simulink model "original_long_instrumented"  (R2026b)
settings: Solver=ode4  StopTime=4  FixedStep=1.0000000000000001e-05
InitFcn:
  | acf_select_actuator(bdroot);
model workspace (MAT data in the model file):
  acfControlVersion = 'force-observer-v1'
  acfImplementation = 'simple'
  acfLayoutVersion = 1
  p : object (value not decoded)
  pCompliant : object (value not decoded)
  pNearContact : object (value not decoded)
  pNoSprings : object (value not decoded)
  pRecommended : object (value not decoded)
symbols that are objects in the model workspace (value not decoded): p
undefined symbols (not defined in the file): DiscIntNeverNeededParam
(part 2 of 3)

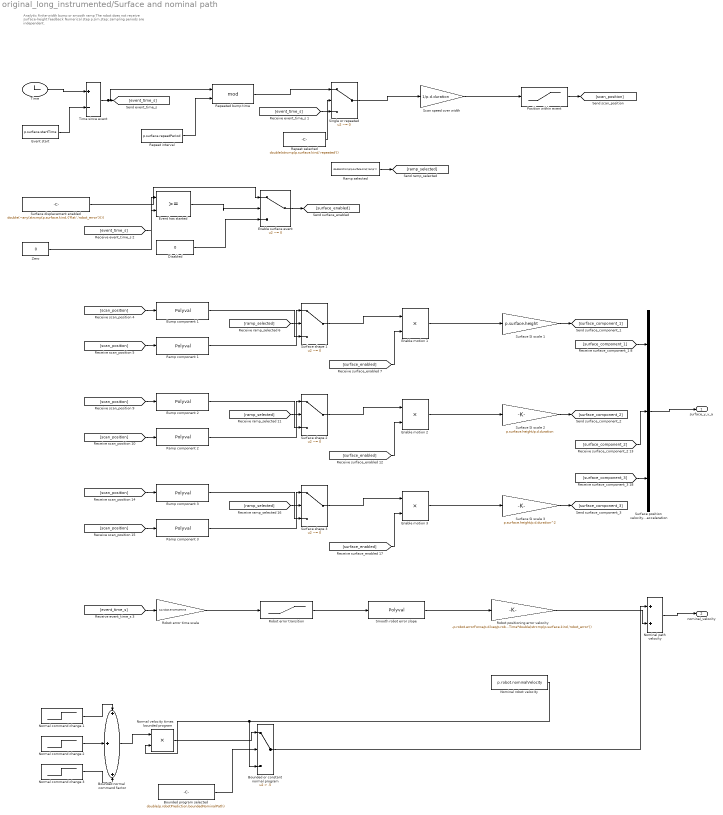
== system original_long_instrumented/Surface and nominal path ==
  note: Analytic finite-width bump or smooth ramp
      | The robot does not receive surface-height feedback
      | Numerical step p.sim.step; sampling periods are independent.
  Bounded normal command factor : Sum  Inputs=+++
  Bounded or constant normal program : Switch  Criteria=u2 > Threshold  Threshold=.5  SaturateOnIntegerOverflow=off  InputSameDT=off
  Bounded program selected : Constant  Value=double(p.robotPrediction.boundedNominalPath)
  Bump component 1 : Polyval  Coefs=[-64 192 -192 64 0 0 0]
  Bump component 2 : Polyval  Coefs=[-384 960 -768 192 0 0]
  Bump component 3 : Polyval  Coefs=[-1920 3840 -2304 384 0]
  Disabled : Constant  Value=0
  Enable motion 1 : Product
  Enable motion 2 : Product
  Enable motion 3 : Product
  Enable surface event : Switch  Criteria=u2 ~= 0  SaturateOnIntegerOverflow=off  InputSameDT=off
  Event has started : RelationalOperator  OutDataTypeStr=boolean  RndMeth=Simplest  InputSameDT=off
  Event start : Constant  Value=p.surface.startTime
  Nominal path velocity : Sum
  Nominal robot velocity : Constant  Value=p.robot.nominalVelocity
  Normal command change 1 : Step  SampleTime=p.robot.sampleTime
  Normal command change 2 : Step  Time=2  FinalValue=-2  SampleTime=p.robot.sampleTime
  Normal command change 3 : Step  Time=3  SampleTime=p.robot.sampleTime
  Normal velocity times bounded program : Product
  Position within event : Saturate  UpperLimit=1  LowerLimit=0
  Ramp component 1 : Polyval  Coefs=[6 -15 10 0 0 0]
  Ramp component 2 : Polyval  Coefs=[30 -60 30 0 0]
  Ramp component 3 : Polyval  Coefs=[120 -180 60 0]
  Ramp selected : Constant  Value=double(strcmp(p.surface.kind,'ramp'))
  Repeat interval : Constant  Value=p.surface.repeatPeriod
  Repeat selected : Constant  Value=double(strcmp(p.surface.kind,'repeated'))
  Repeated bump time : Math  Operator=mod
  Robot error time scale : Gain  Gain=1/p.robot.errorRiseTime
  Robot error transition : Saturate  UpperLimit=1  LowerLimit=0
  Robot positioning error velocity : Gain  Gain=-p.robot.errorForce/p.d.keq/p.robot.errorRiseTime*double(strcmp(p.surface.kind,'robot_error'))
  Scan speed over width : Gain  Gain=1/p.d.duration
  Single or repeated : Switch  Criteria=u2 ~= 0  SaturateOnIntegerOverflow=off  InputSameDT=off
  Smooth robot error slope : Polyval  Coefs=[30 -60 30 0 0]
  Surface SI scale 1 : Gain  Gain=p.surface.height
  Surface SI scale 2 : Gain  Gain=p.surface.height/p.d.duration
  Surface SI scale 3 : Gain  Gain=p.surface.height/p.d.duration^2
  Surface displacement enabled : Constant  Value=double(~any(strcmp(p.surface.kind,{'flat','robot_error'})))
  Surface position velocity acceleration : Mux  Inputs=3
  Surface shape 1 : Switch  Criteria=u2 ~= 0  SaturateOnIntegerOverflow=off  InputSameDT=off
  Surface shape 2 : Switch  Criteria=u2 ~= 0  SaturateOnIntegerOverflow=off  InputSameDT=off
  Surface shape 3 : Switch  Criteria=u2 ~= 0  SaturateOnIntegerOverflow=off  InputSameDT=off
  Time : Clock
  Time since event : Sum  Inputs=+-
  Zero : Constant  Value=0
  surface_y_v_a : Outport
  nominal_velocity : Outport  Port=2
  wires:
  [scan_position] -> Bump component 1/1
  [scan_position] -> Bump component 2/1
  [scan_position] -> Bump component 3/1
  Surface shape 1/1 -> Enable motion 1/1
  [surface_enabled] -> Enable motion 1/2
  Surface shape 2/1 -> Enable motion 2/1
  [surface_enabled] -> Enable motion 2/2
  Surface shape 3/1 -> Enable motion 3/1
  [surface_enabled] -> Enable motion 3/2
  Surface displacement enabled/1 -> Enable surface event/1
  Event has started/1 -> Enable surface event/2
  Disabled/1 -> Enable surface event/3
  [event_time_s] -> Event has started/1
  Zero/1 -> Event has started/2
  Robot positioning error velocity/1 -> Nominal path velocity/2
  Scan speed over width/1 -> Position within event/1
  [scan_position] -> Ramp component 1/1
  [scan_position] -> Ramp component 2/1
  [scan_position] -> Ramp component 3/1
  Time since event/1 -> Repeated bump time/1, [event_time_s]
  Repeat interval/1 -> Repeated bump time/2
  [event_time_s] -> Robot error time scale/1
  Robot error time scale/1 -> Robot error transition/1
  Smooth robot error slope/1 -> Robot positioning error velocity/1
  Single or repeated/1 -> Scan speed over width/1
  Ramp selected/1 -> [ramp_selected]
  Position within event/1 -> [scan_position]
  Surface SI scale 1/1 -> [surface_component_1]
  Surface SI scale 2/1 -> [surface_component_2]
  Surface SI scale 3/1 -> [surface_component_3]
  Enable surface event/1 -> [surface_enabled]
  Repeated bump time/1 -> Single or repeated/1
  Repeat selected/1 -> Single or repeated/2
  [event_time_s] -> Single or repeated/3
  Robot error transition/1 -> Smooth robot error slope/1
  Enable motion 1/1 -> Surface SI scale 1/1
  Enable motion 2/1 -> Surface SI scale 2/1
  Enable motion 3/1 -> Surface SI scale 3/1
  [surface_component_1] -> Surface position velocity acceleration/1
  [surface_component_2] -> Surface position velocity acceleration/2
  [surface_component_3] -> Surface position velocity acceleration/3
  Ramp component 1/1 -> Surface shape 1/1
  [ramp_selected] -> Surface shape 1/2
  Bump component 1/1 -> Surface shape 1/3
  Ramp component 2/1 -> Surface shape 2/1
  [ramp_selected] -> Surface shape 2/2
  Bump component 2/1 -> Surface shape 2/3
  Ramp component 3/1 -> Surface shape 3/1
  [ramp_selected] -> Surface shape 3/2
  Bump component 3/1 -> Surface shape 3/3
  Time/1 -> Time since event/1
  Event start/1 -> Time since event/2
  Surface position velocity acceleration/1 -> surface_y_v_a/1
  Nominal path velocity/1 -> nominal_velocity/1
  Normal command change 1/1 -> Bounded normal command factor/1
  Normal command change 2/1 -> Bounded normal command factor/2
  Normal command change 3/1 -> Bounded normal command factor/3
  Bounded normal command factor/1 -> Normal velocity times bounded program/1
  Nominal robot velocity/1 -> Normal velocity times bounded program/2, Bounded or constant normal program/3
  Normal velocity times bounded program/1 -> Bounded or constant normal program/1
  Bounded program selected/1 -> Bounded or constant normal program/2
  Bounded or constant normal program/1 -> Nominal path velocity/1

== system original_long_instrumented/Surface contact force ==
  Axial reaction : Inport
  Physical surface velocity : Inport  Port=2
  Axial reaction factor : Sum  Inputs=+-
  Friction times slope : Gain  Gain=p.contact.mu
  Lateral reaction : Product  Inputs=**/
  Lateral sign : Gain  Gain=-1
  Normal reaction : Product  Inputs=**/
  Normalizer : Math  Operator=sqrt
  Slope plus friction : Bias  Bias=p.contact.mu  SaturateOnIntegerOverflow=off
  Squared slope : Math  Operator=square
  Squared slope plus one : Bias  Bias=1  SaturateOnIntegerOverflow=off
  Surface slope : Gain  Gain=1/p.surface.scanSpeed
  Unity : Constant
  Velocity component : Selector  InputPortWidth=3  IndexOptions=Index vector (dialog)  Indices=2  OutputSizes=1
  tag scope: actual_contact_slope=global, lateral_contact_N=global, normal_contact_N=global
  wires:
  Physical surface velocity/1 -> Velocity component/1
  Velocity component/1 -> Surface slope/1
  Surface slope/1 -> Squared slope/1, Friction times slope/1, Slope plus friction/1, [actual_contact_slope]
  Squared slope/1 -> Squared slope plus one/1
  Squared slope plus one/1 -> Normalizer/1
  Unity/1 -> Axial reaction factor/1
  Friction times slope/1 -> Axial reaction factor/2
  Axial reaction/1 -> Normal reaction/1
  Normalizer/1 -> Normal reaction/2, Lateral reaction/3
  Axial reaction factor/1 -> Normal reaction/3
  Normal reaction/1 -> Lateral reaction/1, [normal_contact_N]
  Slope plus friction/1 -> Lateral reaction/2
  Lateral reaction/1 -> Lateral sign/1
  Lateral sign/1 -> [lateral_contact_N]

== system original_long_instrumented/Actuator and RABS mechanics/Actuator ==
  Command : Inport
  Gap position velocity : Inport  Port=2
  Spring load : Inport  Port=3
  Ideal position : Subsystem  VariantControl=Ideal position
  Leadscrew : Subsystem  VariantControl=Leadscrew
  Voice coil : Subsystem  VariantControl=Voice coil
  Transmitted force : Outport
  Drive measurements : Outport  Port=2

== system original_long_instrumented/Actuator and RABS mechanics/B to S spring and damper ==
  S position velocity : Inport
  B position velocity : Inport  Port=2
  Rigid reaction : Inport  Port=3
  Compliant or rigid link : VariantSource  VariantControlMode=label  LabelModeActiveChoice=Compliant  VariantControls={Compliant, Rigid}
  Damping : Gain  Gain=p.mechanics.c1
  Endpoint difference : Sum  Inputs=+-
  Preload : Constant  Value=p.d.q10
  Spring and damper force : Sum  Inputs=+++
  Spring displacement and relative velocity : Demux  Outputs=2
  Stiffness : Gain  Gain=p.mechanics.k1
  Spring force : Outport
  wires:
  Spring displacement and relative velocity/2 -> Damping/1
  S position velocity/1 -> Endpoint difference/1
  B position velocity/1 -> Endpoint difference/2
  Preload/1 -> Spring and damper force/1
  Stiffness/1 -> Spring and damper force/2
  Damping/1 -> Spring and damper force/3
  Endpoint difference/1 -> Spring displacement and relative velocity/1
  Spring displacement and relative velocity/1 -> Stiffness/1
  Spring and damper force/1 -> Compliant or rigid link/1
  Rigid reaction/1 -> Compliant or rigid link/2
  Compliant or rigid link/1 -> Spring force/1

== system original_long_instrumented/Actuator and RABS mechanics/Mass A ==
  Actuator force : Inport
  Upper spring force : Inport  Port=2
  Gravity : Constant  Value=p.d.g
  Inverse mass : Gain  Gain=1/p.mechanics.mA
  Net applied force : Sum  Inputs=+-
  Newton acceleration : Sum  Inputs=+-
  Position : Integrator  InitialCondition=p.d.u0
  Position and velocity : Mux  Inputs=2
  Velocity : Integrator
  Position velocity : Outport
  Acceleration : Outport  Port=2
  wires:
  Net applied force/1 -> Inverse mass/1
  Actuator force/1 -> Net applied force/1
  Upper spring force/1 -> Net applied force/2
  Inverse mass/1 -> Newton acceleration/1
  Gravity/1 -> Newton acceleration/2
  Velocity/1 -> Position/1, [velocity_m_s]
  Position/1 -> Position and velocity/1
  [velocity_m_s] -> Position and velocity/2
  Newton acceleration/1 -> Velocity/1, Acceleration/1
  Position and velocity/1 -> Position velocity/1

== system original_long_instrumented/Actuator and RABS mechanics/Mass B ==
  Lower spring force : Inport
  Actuator force : Inport  Port=2
  Gravity : Constant  Value=p.d.g
  Inverse mass : Gain  Gain=1/p.mechanics.mB
  Net applied force : Sum  Inputs=+-
  Newton acceleration : Sum  Inputs=+-
  Position : Integrator
  Position and velocity : Mux  Inputs=2
  Velocity : Integrator
  Position velocity : Outport
  Acceleration : Outport  Port=2
  wires:
  Net applied force/1 -> Inverse mass/1
  Lower spring force/1 -> Net applied force/1
  Actuator force/1 -> Net applied force/2
  Inverse mass/1 -> Newton acceleration/1
  Gravity/1 -> Newton acceleration/2
  Velocity/1 -> Position/1, [velocity_m_s]
  Position/1 -> Position and velocity/1
  [velocity_m_s] -> Position and velocity/2
  Newton acceleration/1 -> Velocity/1, Acceleration/1
  Position and velocity/1 -> Position velocity/1

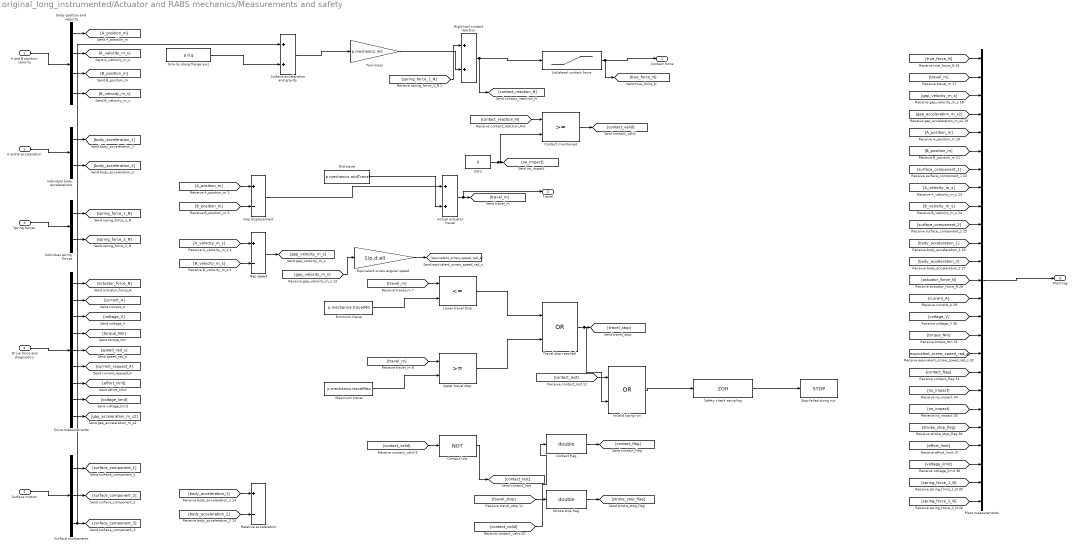
== system original_long_instrumented/Actuator and RABS mechanics/Measurements and safety ==
  A and B position velocity : Inport
  A and B acceleration : Inport  Port=2
  Spring forces : Inport  Port=3
  Drive force and diagnostics : Inport  Port=4
  Surface motion : Inport  Port=5
  Actual actuator travel : Sum
  Body position and velocity : Demux
  Contact flag : DataTypeConversion  OutDataTypeStr=double  SaturateOnIntegerOverflow=off  RndMeth=Floor
  Contact lost : Logic  Operator=NOT  AllPortsSameDT=off  OutDataTypeStr=boolean
  Contact maintained : RelationalOperator  OutDataTypeStr=boolean  RndMeth=Simplest  InputSameDT=off
  Drive measurements : Demux  Outputs=9
  Equivalent screw angular speed : Gain  Gain=1/p.d.ell
  Gap displacement : Sum  Inputs=+-
  Gap speed : Sum  Inputs=+-
  Gravity along flange axis : Constant  Value=p.d.g
  Individual body accelerations : Demux  Outputs=2
  Individual spring forces : Demux  Outputs=2
  Invalid sizing run : Logic  Operator=OR  AllPortsSameDT=off  OutDataTypeStr=boolean
  Lower travel stop : RelationalOperator  Operator=<=  OutDataTypeStr=boolean  RndMeth=Simplest  InputSameDT=off
  Maximum travel : Constant  Value=p.mechanics.travelMax
  Mid travel : Constant  Value=p.mechanics.midTravel
  Minimum travel : Constant  Value=p.mechanics.travelMin
  Plant measurements : Mux  Inputs=25
  Relative acceleration : Sum  Inputs=+-
  Rigid tool contact reaction : Sum
  Safety check sampling : ZeroOrderHold  SampleTime=p.sim.step
  Stop failed sizing run : Stop
  Stroke stop flag : DataTypeConversion  OutDataTypeStr=double  SaturateOnIntegerOverflow=off  RndMeth=Floor
  Surface acceleration and gravity : Sum
  Surface components : Demux  Outputs=3
  Tool mass : Gain  Gain=p.mechanics.mS
  Travel stop reached : Logic  Operator=OR  AllPortsSameDT=off  OutDataTypeStr=boolean
  Unilateral contact force : Saturate  UpperLimit=inf  LowerLimit=0
  Upper travel stop : RelationalOperator  OutDataTypeStr=boolean  RndMeth=Simplest  InputSameDT=off
  Zero : Constant  Value=0
  Contact force : Outport
  Travel : Outport  Port=2
  Plant log : Outport  Port=3
  wires:
  Gap displacement/1 -> Actual actuator travel/1
  Mid travel/1 -> Actual actuator travel/2
  A and B position velocity/1 -> Body position and velocity/1
  [contact_valid] -> Contact flag/1
  [contact_valid] -> Contact lost/1
  [contact_reaction_N] -> Contact maintained/1
  Zero/1 -> Contact maintained/2, [no_impact]
  Drive force and diagnostics/1 -> Drive measurements/1
  [gap_velocity_m_s] -> Equivalent screw angular speed/1
  [A_position_m] -> Gap displacement/1
  [B_position_m] -> Gap displacement/2
  [A_velocity_m_s] -> Gap speed/1
  [B_velocity_m_s] -> Gap speed/2
  A and B acceleration/1 -> Individual body accelerations/1
  Spring forces/1 -> Individual spring forces/1
  [contact_lost] -> Invalid sizing run/1
  Travel stop reached/1 -> Invalid sizing run/2, [travel_stop]
  [travel_m] -> Lower travel stop/1
  Minimum travel/1 -> Lower travel stop/2
  [true_force_N] -> Plant measurements/1
  [travel_m] -> Plant measurements/2
  [gap_velocity_m_s] -> Plant measurements/3
  [gap_acceleration_m_s2] -> Plant measurements/4
  [A_position_m] -> Plant measurements/5
  [B_position_m] -> Plant measurements/6
  [surface_component_1] -> Plant measurements/7
  [A_velocity_m_s] -> Plant measurements/8
  [B_velocity_m_s] -> Plant measurements/9
  [surface_component_2] -> Plant measurements/10
  [body_acceleration_1] -> Plant measurements/11
  [body_acceleration_2] -> Plant measurements/12
  [actuator_force_N] -> Plant measurements/13
  [current_A] -> Plant measurements/14
  [voltage_V] -> Plant measurements/15
  [torque_Nm] -> Plant measurements/16
  [equivalent_screw_speed_rad_s] -> Plant measurements/17
  [contact_flag] -> Plant measurements/18
  [no_impact] -> Plant measurements/19
  [no_impact] -> Plant measurements/20
  [stroke_stop_flag] -> Plant measurements/21
  [effort_limit] -> Plant measurements/22
  [voltage_limit] -> Plant measurements/23
  [spring_force_1_N] -> Plant measurements/24
  [spring_force_2_N] -> Plant measurements/25
  [body_acceleration_1] -> Relative acceleration/1
  [body_acceleration_2] -> Relative acceleration/2
  [spring_force_1_N] -> Rigid tool contact reaction/1
  Tool mass/1 -> Rigid tool contact reaction/2
  Invalid sizing run/1 -> Safety check sampling/1
  Body position and velocity/1 -> [A_position_m]
  Body position and velocity/2 -> [A_velocity_m_s]
  Body position and velocity/3 -> [B_position_m]
  Body position and velocity/4 -> [B_velocity_m_s]
  Drive measurements/1 -> [actuator_force_N]
  Individual body accelerations/1 -> [body_acceleration_1]
  Individual body accelerations/2 -> [body_acceleration_2]
  Contact flag/1 -> [contact_flag]
  Contact lost/1 -> [contact_lost]
  Rigid tool contact reaction/1 -> [contact_reaction_N], Unilateral contact force/1
  Contact maintained/1 -> [contact_valid]
  Drive measurements/2 -> [current_A]
  Drive measurements/6 -> [current_request_A]
  Drive measurements/7 -> [effort_limit]
  Equivalent screw angular speed/1 -> [equivalent_screw_speed_rad_s]
  Drive measurements/9 -> [gap_acceleration_m_s2]
  Gap speed/1 -> [gap_velocity_m_s]
  Drive measurements/5 -> [speed_rad_s]
  Individual spring forces/1 -> [spring_force_1_N]
  Individual spring forces/2 -> [spring_force_2_N]
  Stroke stop flag/1 -> [stroke_stop_flag]
  Surface components/1 -> [surface_component_1]
  Surface components/2 -> [surface_component_2]
  Surface components/3 -> [surface_component_3], Surface acceleration and gravity/1
  Drive measurements/4 -> [torque_Nm]
  Actual actuator travel/1 -> [travel_m], Travel/1
  Unilateral contact force/1 -> [true_force_N], Contact force/1
  Drive measurements/3 -> [voltage_V]
  Drive measurements/8 -> [voltage_limit]
  Safety check sampling/1 -> Stop failed sizing run/1
  [travel_stop] -> Stroke stop flag/1
  Gravity along flange axis/1 -> Surface acceleration and gravity/2
  Surface motion/1 -> Surface components/1
  Surface acceleration and gravity/1 -> Tool mass/1
  Lower travel stop/1 -> Travel stop reached/1
  Upper travel stop/1 -> Travel stop reached/2
  [travel_m] -> Upper travel stop/1
  Maximum travel/1 -> Upper travel stop/2
  Plant measurements/1 -> Plant log/1

== system original_long_instrumented/Actuator and RABS mechanics/R to A spring and damper ==
  A position velocity : Inport
  R position velocity : Inport  Port=2
  Rigid reaction : Inport  Port=3
  Compliant or rigid link : VariantSource  VariantControlMode=label  LabelModeActiveChoice=Rigid  VariantControls={Compliant, Rigid}
  Damping : Gain  Gain=p.mechanics.c2
  Endpoint difference : Sum  Inputs=+-
  Preload : Constant  Value=p.d.q20
  Spring and damper force : Sum  Inputs=+++
  Spring displacement and relative velocity : Demux  Outputs=2
  Stiffness : Gain  Gain=p.mechanics.k2
  Spring force : Outport
  wires:
  Spring displacement and relative velocity/2 -> Damping/1
  A position velocity/1 -> Endpoint difference/1
  R position velocity/1 -> Endpoint difference/2
  Preload/1 -> Spring and damper force/1
  Stiffness/1 -> Spring and damper force/2
  Damping/1 -> Spring and damper force/3
  Endpoint difference/1 -> Spring displacement and relative velocity/1
  Spring displacement and relative velocity/1 -> Stiffness/1
  Spring and damper force/1 -> Compliant or rigid link/1
  Rigid reaction/1 -> Compliant or rigid link/2
  Compliant or rigid link/1 -> Spring force/1

== system original_long_instrumented/Contact force measurement/Contact force reconstruction ==
  raw_cell_error_N : Inport
  Cell error to deviation : Gain  Gain=-1
  Compensated axial reaction : Sum
  Compensated lateral reaction : Sum
  Downstream X inertia : Gain  Gain=p.sensor.distalMass_model_kg
  Downstream Z inertia : Gain  Gain=p.sensor.distalMass_model_kg
  Tared axial cell force : Bias  Bias=p.force.reference  SaturateOnIntegerOverflow=off
  axial_contact_N : Outport
  lateral_contact_N : Outport  Port=2
  tag scope: inertial_axial_contact_N=global, inertial_lateral_contact_N=global
  wires:
  Compensated axial reaction/1 -> axial_contact_N/1, [inertial_axial_contact_N]
  Tared axial cell force/1 -> Compensated axial reaction/1
  Downstream Z inertia/1 -> Compensated axial reaction/2
  Compensated lateral reaction/1 -> lateral_contact_N/1, [inertial_lateral_contact_N]
  Cell error to deviation/1 -> Tared axial cell force/1
  [measured_S_acceleration_z] -> Downstream Z inertia/1
  [measured_lateral_contact_N] -> Compensated lateral reaction/1
  Downstream X inertia/1 -> Compensated lateral reaction/2
  raw_cell_error_N/1 -> Cell error to deviation/1
  [measured_S_acceleration_x] -> Downstream X inertia/1

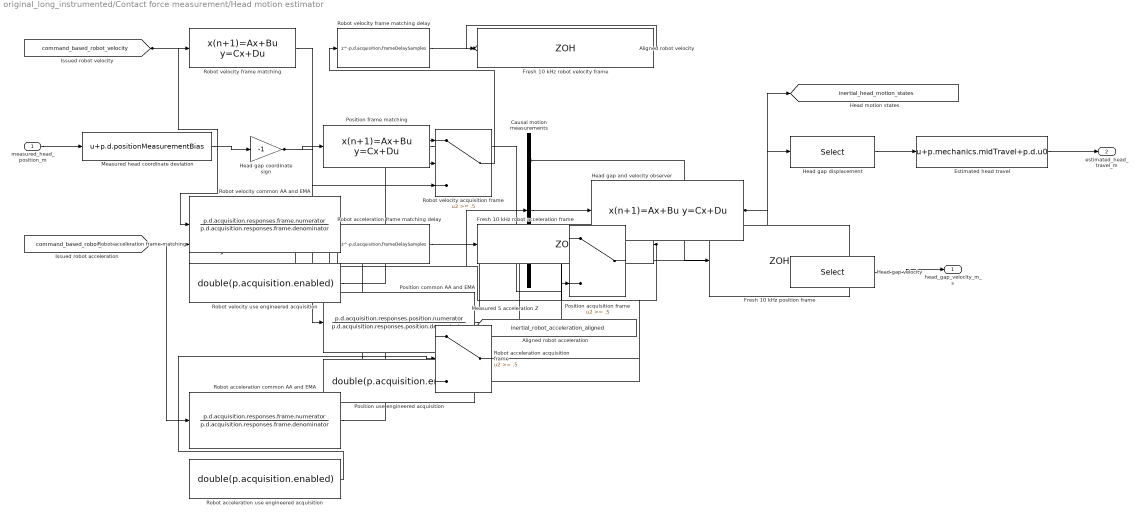
== system original_long_instrumented/Contact force measurement/Head motion estimator ==
  measured_head_position_m : Inport
  Causal motion measurements : Mux  Inputs=3
  Estimated head travel : Bias  Bias=p.mechanics.midTravel+p.d.u0  SaturateOnIntegerOverflow=off
  Fresh 10 kHz position frame : ZeroOrderHold  SampleTime=p.force.sampleTime
  Fresh 10 kHz robot acceleration frame : ZeroOrderHold  SampleTime=p.force.sampleTime
  Fresh 10 kHz robot velocity frame : ZeroOrderHold  SampleTime=p.force.sampleTime
  Head gap and velocity observer : DiscreteStateSpace  A=p.d.toolMotionObserver.A  B=p.d.toolMotionObserver.B  C=p.d.toolMotionObserver.C  D=p.d.toolMotionObserver.D  InitialCondition=zeros(2,1)  SampleTime=p.force.sampleTime
  Head gap coordinate sign : Gain  Gain=-1
  Head gap displacement : Selector  InputPortWidth=2  IndexOptions=Index vector (dialog)  Indices=1  OutputSizes=1
  Head gap velocity : Selector  InputPortWidth=2  IndexOptions=Index vector (dialog)  Indices=2  OutputSizes=1
  Measured head coordinate deviation : Bias  Bias=p.d.positionMeasurementBias  SaturateOnIntegerOverflow=off
  Position acquisition frame : Switch  Threshold=.5  SaturateOnIntegerOverflow=off  InputSameDT=off
  Position common AA and EMA : DiscreteTransferFcn  Numerator=p.d.acquisition.responses.position.numerator  Denominator=p.d.acquisition.responses.position.denominator  InitialStates=(0)*p.d.acquisition.responses.position.steadyStatePerUnitInput  SampleTime=p.sensor.sampleTime
  Position frame matching : DiscreteStateSpace  A=exp(-p.sensor.sampleTime/p.sensor.filterTime)  B=1-exp(-p.sensor.sampleTime/p.sensor.filterTime)  C=exp(-p.sensor.sampleTime/p.sensor.filterTime)  D=1-exp(-p.sensor.sampleTime/p.sensor.filterTime)  SampleTime=p.sensor.sampleTime
  Position use engineered acquisition : Constant  Value=double(p.acquisition.enabled)
  Robot acceleration acquisition frame : Switch  Threshold=.5  SaturateOnIntegerOverflow=off  InputSameDT=off
  Robot acceleration common AA and EMA : DiscreteTransferFcn  Numerator=p.d.acquisition.responses.frame.numerator  Denominator=p.d.acquisition.responses.frame.denominator  InitialStates=(0)*p.d.acquisition.responses.frame.steadyStatePerUnitInput  SampleTime=p.sensor.sampleTime
  Robot acceleration frame matching : DiscreteStateSpace  A=exp(-p.sensor.sampleTime/p.sensor.filterTime)  B=1-exp(-p.sensor.sampleTime/p.sensor.filterTime)  C=exp(-p.sensor.sampleTime/p.sensor.filterTime)  D=1-exp(-p.sensor.sampleTime/p.sensor.filterTime)  SampleTime=p.sensor.sampleTime
  Robot acceleration frame matching delay : Delay  DelayLength=p.d.acquisition.frameDelaySamples  InitialCondition=0  SampleTime=p.sensor.sampleTime
  Robot acceleration use engineered acquisition : Constant  Value=double(p.acquisition.enabled)
  Robot velocity acquisition frame : Switch  Threshold=.5  SaturateOnIntegerOverflow=off  InputSameDT=off
  Robot velocity common AA and EMA : DiscreteTransferFcn  Numerator=p.d.acquisition.responses.frame.numerator  Denominator=p.d.acquisition.responses.frame.denominator  InitialStates=(0)*p.d.acquisition.responses.frame.steadyStatePerUnitInput  SampleTime=p.sensor.sampleTime
  Robot velocity frame matching : DiscreteStateSpace  A=exp(-p.sensor.sampleTime/p.sensor.filterTime)  B=1-exp(-p.sensor.sampleTime/p.sensor.filterTime)  C=exp(-p.sensor.sampleTime/p.sensor.filterTime)  D=1-exp(-p.sensor.sampleTime/p.sensor.filterTime)  SampleTime=p.sensor.sampleTime
  Robot velocity frame matching delay : Delay  DelayLength=p.d.acquisition.frameDelaySamples  InitialCondition=0  SampleTime=p.sensor.sampleTime
  Robot velocity use engineered acquisition : Constant  Value=double(p.acquisition.enabled)
  head_gap_velocity_m_s : Outport
  estimated_head_travel_m : Outport  Port=2
  tag scope: inertial_head_motion_states=global, inertial_robot_acceleration_aligned=global, inertial_robot_velocity_aligned=global
  wires:
  Estimated head travel/1 -> estimated_head_travel_m/1
  measured_head_position_m/1 -> Measured head coordinate deviation/1
  Head gap velocity/1 -> head_gap_velocity_m_s/1
  [command_based_robot_velocity] -> Robot velocity frame matching/1, Robot velocity common AA and EMA/1
  Measured head coordinate deviation/1 -> Head gap coordinate sign/1
  [command_based_robot_acceleration] -> Robot acceleration frame matching/1, Robot acceleration common AA and EMA/1
  Head gap coordinate sign/1 -> Position frame matching/1, Position common AA and EMA/1
  Causal motion measurements/1 -> Head gap and velocity observer/1
  Head gap displacement/1 -> Estimated head travel/1
  Head gap and velocity observer/1 -> Head gap displacement/1, Head gap velocity/1, [inertial_head_motion_states]
  [measured_S_acceleration_z] -> Causal motion measurements/3
  Position common AA and EMA/1 -> Position acquisition frame/1
  Position use engineered acquisition/1 -> Position acquisition frame/2
  Position frame matching/1 -> Position acquisition frame/3
  Position acquisition frame/1 -> Fresh 10 kHz position frame/1
  Fresh 10 kHz position frame/1 -> Causal motion measurements/1
  Robot acceleration common AA and EMA/1 -> Robot acceleration acquisition frame/1
  Robot acceleration use engineered acquisition/1 -> Robot acceleration acquisition frame/2
  Robot acceleration frame matching/1 -> Robot acceleration acquisition frame/3
  Robot acceleration acquisition frame/1 -> Robot acceleration frame matching delay/1
  Robot acceleration frame matching delay/1 -> Fresh 10 kHz robot acceleration frame/1
  Fresh 10 kHz robot acceleration frame/1 -> [inertial_robot_acceleration_aligned], Causal motion measurements/2
  Robot velocity common AA and EMA/1 -> Robot velocity acquisition frame/1
  Robot velocity use engineered acquisition/1 -> Robot velocity acquisition frame/2
  Robot velocity frame matching/1 -> Robot velocity acquisition frame/3
  Robot velocity acquisition frame/1 -> Robot velocity frame matching delay/1
  Robot velocity frame matching delay/1 -> Fresh 10 kHz robot velocity frame/1
  Fresh 10 kHz robot velocity frame/1 -> [inertial_robot_velocity_aligned]

== system original_long_instrumented/Contact force measurement/Normal force projection ==
  Compensated axial force : Inport
  Compensated lateral force : Inport  Port=2
  Head gap velocity : Inport  Port=3
  Axial reference deviation : Bias  Bias=-p.force.reference  SaturateOnIntegerOverflow=off
  Causal surface direction : Gain  Gain=1/p.contact.commandedScanSpeed_m_s
  Estimated S velocity : Sum  Inputs=+-
  Lateral projection : Product  Inputs=**
  Measured drag audit vector : Mux  Inputs=3
  Measured drag geometry : Subsystem
  Measured drag geometry selected : Constant  Value=double(strcmp(p.contact.geometryMode,'measured_drag_ratio'))
  Measured drag native log : ToWorkspace  VariableName=measured_drag_log  SaveFormat=Timeseries  SampleTime=-1
  Measured drag native sample 1 : ZeroOrderHold  SampleTime=p.sim.step
  Measured drag native sample 2 : ZeroOrderHold  SampleTime=p.sim.step
  Measured drag native sample 3 : ZeroOrderHold  SampleTime=p.sim.step
  Measured normal force : Product  Inputs=*/
  Measured normal force deviation : Bias  Bias=-p.force.reference  SaturateOnIntegerOverflow=off
  Normal projection numerator : Sum  Inputs=+-
  Normal reference projection : Gain  Gain=p.force.reference
  Normalizer : Math  Operator=sqrt
  Requested axial force : Sum
  Select axial force geometry request : Switch  Threshold=.5  SaturateOnIntegerOverflow=off  InputSameDT=off
  Squared slope : Math  Operator=square
  Squared slope plus one : Bias  Bias=1  SaturateOnIntegerOverflow=off
  normal_force_deviation_N : Outport
  axial_reference_deviation_N : Outport  Port=2
  tag scope: estimated_contact_slope=global, estimated_normal_contact_N=global, requested_axial_contact_N=global
  wires:
  Axial reference deviation/1 -> axial_reference_deviation_N/1
  Measured normal force deviation/1 -> normal_force_deviation_N/1
  Head gap velocity/1 -> Estimated S velocity/2
  [inertial_robot_velocity_aligned] -> Estimated S velocity/1
  Squared slope/1 -> Squared slope plus one/1
  Compensated lateral force/1 -> Lateral projection/1, Measured drag geometry/2(reconstructed_Rx_N)
  Lateral projection/1 -> Normal projection numerator/2, Requested axial force/2
  Estimated S velocity/1 -> Causal surface direction/1
  Compensated axial force/1 -> Normal projection numerator/1, Measured drag geometry/1(reconstructed_Rz_N)
  Normal reference projection/1 -> Requested axial force/1
  Normal projection numerator/1 -> Measured normal force/1
  Normalizer/1 -> Measured normal force/2, Normal reference projection/1, Measured drag geometry/5(normalizer)
  Causal surface direction/1 -> Squared slope/1, [estimated_contact_slope], Lateral projection/2, Measured drag geometry/3(estimated_slope)
  Squared slope plus one/1 -> Normalizer/1
  Measured normal force/1 -> Measured normal force deviation/1, [estimated_normal_contact_N], Measured drag geometry/4(estimated_normal_N)
  Measured drag geometry/1(requested_Rz_N) -> Select axial force geometry request/1
  Measured drag geometry selected/1 -> Select axial force geometry request/2
  Requested axial force/1 -> Select axial force geometry request/3
  Select axial force geometry request/1 -> Axial reference deviation/1, [requested_axial_contact_N]
  Measured drag geometry/2(filtered_drag_ratio) -> Measured drag native sample 1/1
  Measured drag native sample 1/1 -> Measured drag audit vector/1
  Measured drag geometry/3(bounded_raw_drag_ratio) -> Measured drag native sample 2/1
  Measured drag native sample 2/1 -> Measured drag audit vector/2
  Measured drag geometry/4(drag_estimate_valid) -> Measured drag native sample 3/1
  Measured drag native sample 3/1 -> Measured drag audit vector/3
  Measured drag audit vector/1 -> Measured drag native log/1

== system original_long_instrumented/Force controller/Coil PI and PID ==
  error_N : Inport
  measured_travel_m : Inport  Port=2
  Current limits : Saturate  UpperLimit=p.coil.peakCurrent  LowerLimit=-p.coil.peakCurrent
  Current saturation error : Sum  Inputs=+-
  Flat holding current : Constant  Value=(p.force.reference-(p.uncertainty.massB_model_kg+p.sensor.distalMass_model_kg)*p.d.g)/p.uncertainty.forceConstant_model_N_A
  Integral anti windup : Gain  Gain=-p.force.antiWindupRate/p.inertial.forceKi
  Lower spring inverse feedforward : Subsystem
  Measured motion feedforward : Subsystem
  Normal force PI and PID : Subsystem
  Optional structural-mode current notch : DiscreteTransferFcn  Numerator=p.d.currentNotch.numerator  Denominator=p.d.currentNotch.denominator  InitialStates=p.d.currentNotch.initialStates  SampleTime=p.force.sampleTime
  PI PID and feedforward current : Sum  Inputs=++++++
  command : Outport
  estimated_travel_m : Outport  Port=2
  estimated_force_error_N : Outport  Port=3
  wires:
  measured_travel_m/1 -> estimated_travel_m/1
  Optional structural-mode current notch/1 -> Current limits/1, Current saturation error/2
  Integral anti windup/1 -> Normal force PI and PID/2(anti_windup)
  Current limits/1 -> command/1, Current saturation error/1
  PI PID and feedforward current/1 -> Optional structural-mode current notch/1
  Current saturation error/1 -> Integral anti windup/1
  error_N/1 -> estimated_force_error_N/1, Normal force PI and PID/1(error_N)
  Flat holding current/1 -> PI PID and feedforward current/1
  Normal force PI and PID/1(feedback_current_A) -> PI PID and feedforward current/2
  Measured motion feedforward/1(acceleration_current_A) -> PI PID and feedforward current/3
  Measured motion feedforward/2(geometry_current_A) -> PI PID and feedforward current/4
  Measured motion feedforward/3(friction_current_A) -> PI PID and feedforward current/5
  Lower spring inverse feedforward/1(extra_current_A) -> PI PID and feedforward current/6

== system original_long_instrumented/Force controller/Drive PI and PID ==
  note: Sampled PI + anti-windup
      | Coil: amperes; screw: rad/s; ideal: gap in metres
      | Numerical step p.sim.step; sampling periods are independent.
  note: PI / FILTERED PID
      | Kp, Ki, Kd and derivative-filter time are ordinary parameters.
      | Kd = 0 disables derivative action. Voice-coil strategy chooses this page or the observer.
  error_N : Inport
  measured_travel_m : Inport  Port=2
  Actuator command limits : Saturate  UpperLimit=p.d.commandMax  LowerLimit=p.d.commandMin
  Anti windup : Gain  Gain=p.force.antiWindupRate
  Derivative gain : Gain  Gain=p.d.forceKd*double(strcmp(p.coil.strategy,'pid'))
  Filtered force derivative : DiscreteTransferFcn  Numerator=(1-exp(-p.force.sampleTime/p.d.derivativeFilter))/p.force.sampleTime*[1 -1]  Denominator=[1 -exp(-p.force.sampleTime/p.d.derivativeFilter)]  SampleTime=p.force.sampleTime
  Force controller sampling : ZeroOrderHold  SampleTime=p.force.sampleTime
  Holding command : Constant  Value=p.d.forceFeedforward
  Integral action : DiscreteIntegrator  SampleTime=p.force.sampleTime  ICPrevOutput=DiscIntNeverNeededParam  ICPrevScaledInput=DiscIntNeverNeededParam
  Integral gain : Gain  Gain=p.d.forceKi
  Integral input : Sum
  PI plus holding command : Sum  Inputs=++++
  Proportional gain : Gain  Gain=p.d.forceKp
  Saturation error : Sum  Inputs=+-
  command : Outport
  estimated_travel_m : Outport  Port=2
  estimated_force_error_N : Outport  Port=3
  wires:
  Actuator command limits/1 -> [limited_command], command/1
  Integral action/1 -> [integral_command]
  PI plus holding command/1 -> Actuator command limits/1, [raw_command]
  Integral input/1 -> Integral action/1
  Holding command/1 -> PI plus holding command/3
  error_N/1 -> estimated_force_error_N/1, Force controller sampling/1
  measured_travel_m/1 -> estimated_travel_m/1
  [force_error_N] -> Integral gain/1
  [force_error_N] -> Filtered force derivative/1
  Derivative gain/1 -> [derivative_command]
  Saturation error/1 -> Anti windup/1
  [limited_command] -> Saturation error/1
  Force controller sampling/1 -> Proportional gain/1, [force_error_N]
  Anti windup/1 -> [tracking_correction]
  [raw_command] -> Saturation error/2
  Integral gain/1 -> Integral input/1
  [derivative_command] -> PI plus holding command/4
  [integral_command] -> PI plus holding command/2
  Filtered force derivative/1 -> Derivative gain/1
  [tracking_correction] -> Integral input/2
  Proportional gain/1 -> PI plus holding command/1

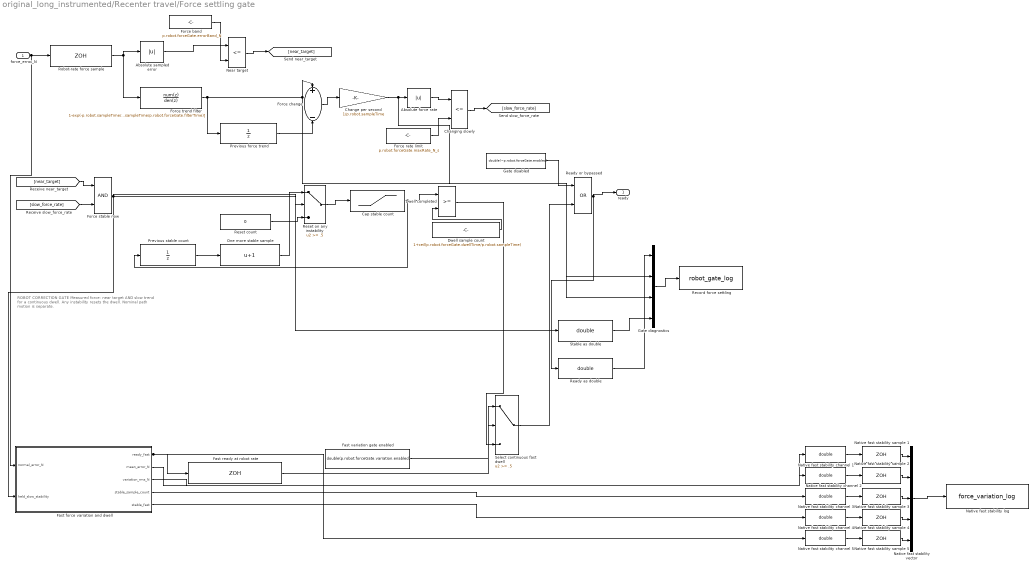
== system original_long_instrumented/Recenter travel/Force settling gate ==
  note: ROBOT CORRECTION GATE
      | Measured force: near target AND slow trend for a continuous dwell.
      | Any instability resets the dwell. Nominal path motion is separate.
  force_error_N : Inport
  Absolute force rate : Abs  SaturateOnIntegerOverflow=off
  Absolute sampled error : Abs  SaturateOnIntegerOverflow=off
  Cap stable count : Saturate  UpperLimit=1+ceil(p.robot.forceGate.dwellTime/p.robot.sampleTime)  LowerLimit=0
  Change per second : Gain  Gain=1/p.robot.sampleTime
  Changing slowly : RelationalOperator  Operator=<=  OutDataTypeStr=boolean  RndMeth=Simplest  InputSameDT=off
  Dwell completed : RelationalOperator  OutDataTypeStr=boolean  RndMeth=Simplest  InputSameDT=off
  Dwell sample count : Constant  Value=1+ceil(p.robot.forceGate.dwellTime/p.robot.sampleTime)
  Fast force variation and dwell : Subsystem
  Fast ready at robot rate : ZeroOrderHold  SampleTime=p.robot.sampleTime
  Fast variation gate enabled : Constant  Value=double(p.robot.forceGate.variation.enabled)
  Force band : Constant  Value=p.robot.forceGate.errorBand_N
  Force change : Sum  Inputs=+-
  Force rate limit : Constant  Value=p.robot.forceGate.maxRate_N_s
  Force stable now : Logic  AllPortsSameDT=off  OutDataTypeStr=boolean
  Force trend filter : DiscreteTransferFcn  Numerator=1-exp(-p.robot.sampleTime/p.robot.forceGate.filterTime)  Denominator=[1 -exp(-p.robot.sampleTime/p.robot.forceGate.filterTime)]  SampleTime=p.robot.sampleTime
  Gate diagnostics : Mux
  Gate disabled : Constant  Value=double(~p.robot.forceGate.enabled)
  Native fast stability channel {1..5} (5 alike) : DataTypeConversion  OutDataTypeStr=double  SaturateOnIntegerOverflow=off  RndMeth=Floor
  Native fast stability log : ToWorkspace  VariableName=force_variation_log  SaveFormat=Timeseries  SampleTime=-1
  Native fast stability sample {1..5} (5 alike) : ZeroOrderHold  SampleTime=p.sim.step
  Native fast stability vector : Mux  Inputs=5
  Near target : RelationalOperator  Operator=<=  OutDataTypeStr=boolean  RndMeth=Simplest  InputSameDT=off
  One more stable sample : Bias  Bias=1  SaturateOnIntegerOverflow=off
  Previous force trend : UnitDelay  SampleTime=p.robot.sampleTime
  Previous stable count : UnitDelay  SampleTime=p.robot.sampleTime
  Ready as double : DataTypeConversion  OutDataTypeStr=double  SaturateOnIntegerOverflow=off  RndMeth=Floor
  Ready or bypassed : Logic  Operator=OR  AllPortsSameDT=off  OutDataTypeStr=boolean
  Record force settling : ToWorkspace  VariableName=robot_gate_log  SaveFormat=Timeseries  SampleTime=p.robot.sampleTime
  Reset count : Constant  Value=0
  Reset on any instability : Switch  Threshold=.5  SaturateOnIntegerOverflow=off  InputSameDT=off
  Robot-rate force sample : ZeroOrderHold  SampleTime=p.robot.sampleTime
  Select continuous fast dwell : Switch  Threshold=.5  SaturateOnIntegerOverflow=off  InputSameDT=off
  Stable as double : DataTypeConversion  OutDataTypeStr=double  SaturateOnIntegerOverflow=off  RndMeth=Floor
  ready : Outport
  wires:
  force_error_N/1 -> Robot-rate force sample/1, Fast force variation and dwell/1(normal_error_N)
  Robot-rate force sample/1 -> Absolute sampled error/1, Force trend filter/1
  Absolute sampled error/1 -> Near target/1
  Force band/1 -> Near target/2
  Near target/1 -> [near_target]
  Force trend filter/1 -> Force change/1, Gate diagnostics/2, Previous force trend/1
  Previous force trend/1 -> Force change/2
  Force change/1 -> Change per second/1
  Change per second/1 -> Absolute force rate/1, Gate diagnostics/3
  Absolute force rate/1 -> Changing slowly/1
  Force rate limit/1 -> Changing slowly/2
  Changing slowly/1 -> [slow_force_rate]
  [near_target] -> Force stable now/1
  [slow_force_rate] -> Force stable now/2
  Previous stable count/1 -> One more stable sample/1
  One more stable sample/1 -> Reset on any instability/1
  Force stable now/1 -> Reset on any instability/2, Stable as double/1, Fast force variation and dwell/2(held_slow_stability)
  Reset count/1 -> Reset on any instability/3
  Reset on any instability/1 -> Cap stable count/1
  Cap stable count/1 -> Previous stable count/1, Dwell completed/1
  Dwell sample count/1 -> Dwell completed/2
  Gate disabled/1 -> Ready or bypassed/1
  Ready or bypassed/1 -> ready/1, Ready as double/1
  Gate diagnostics/1 -> Record force settling/1
  Ready as double/1 -> Gate diagnostics/1
  Stable as double/1 -> Gate diagnostics/4
  Fast force variation and dwell/1(ready_fast) -> Fast ready at robot rate/1, Native fast stability channel 5/1
  Fast ready at robot rate/1 -> Select continuous fast dwell/1
  Fast variation gate enabled/1 -> Select continuous fast dwell/2
  Dwell completed/1 -> Select continuous fast dwell/3
  Select continuous fast dwell/1 -> Ready or bypassed/2
  Fast force variation and dwell/2(mean_error_N) -> Native fast stability channel 1/1
  Native fast stability channel 1/1 -> Native fast stability sample 1/1
  Native fast stability sample 1/1 -> Native fast stability vector/1
  Fast force variation and dwell/3(variation_rms_N) -> Native fast stability channel 2/1
  Native fast stability channel 2/1 -> Native fast stability sample 2/1
  Native fast stability sample 2/1 -> Native fast stability vector/2
  Fast force variation and dwell/4(stable_sample_count) -> Native fast stability channel 3/1
  Native fast stability channel 3/1 -> Native fast stability sample 3/1
  Native fast stability sample 3/1 -> Native fast stability vector/3
  Fast force variation and dwell/5(stable_fast) -> Native fast stability channel 4/1
  Native fast stability channel 4/1 -> Native fast stability sample 4/1
  Native fast stability sample 4/1 -> Native fast stability vector/4
  Native fast stability channel 5/1 -> Native fast stability sample 5/1
  Native fast stability sample 5/1 -> Native fast stability vector/5
  Native fast stability vector/1 -> Native fast stability log/1

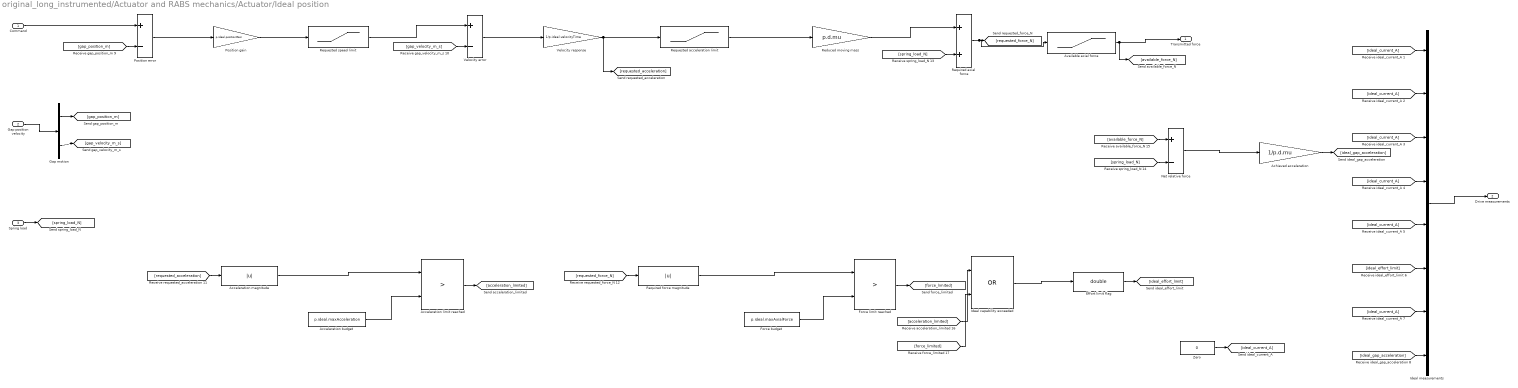
== system original_long_instrumented/Actuator and RABS mechanics/Actuator/Ideal position ==
  Command : Inport
  Gap position velocity : Inport  Port=2
  Spring load : Inport  Port=3
  Acceleration budget : Constant  Value=p.ideal.maxAcceleration
  Acceleration limit reached : RelationalOperator  Operator=>  OutDataTypeStr=boolean  RndMeth=Simplest  InputSameDT=off
  Acceleration magnitude : Abs  SaturateOnIntegerOverflow=off
  Achieved acceleration : Gain  Gain=1/p.d.mu
  Available axial force : Saturate  UpperLimit=p.ideal.maxAxialForce  LowerLimit=-p.ideal.maxAxialForce
  Effort limit flag : DataTypeConversion  OutDataTypeStr=double  SaturateOnIntegerOverflow=off  RndMeth=Floor
  Force budget : Constant  Value=p.ideal.maxAxialForce
  Force limit reached : RelationalOperator  Operator=>  OutDataTypeStr=boolean  RndMeth=Simplest  InputSameDT=off
  Gap motion : Demux  Outputs=2
  Ideal capability exceeded : Logic  Operator=OR  AllPortsSameDT=off  OutDataTypeStr=boolean
  Ideal measurements : Mux  Inputs=8
  Net relative force : Sum  Inputs=+-
  Position error : Sum  Inputs=+-
  Position gain : Gain  Gain=p.ideal.positionGain
  Reduced moving mass : Gain  Gain=p.d.mu
  Requested acceleration limit : Saturate  UpperLimit=p.ideal.maxAcceleration  LowerLimit=-p.ideal.maxAcceleration
  Requested speed limit : Saturate  UpperLimit=p.ideal.maxSpeed  LowerLimit=-p.ideal.maxSpeed
  Required axial force : Sum
  Required force magnitude : Abs  SaturateOnIntegerOverflow=off
  Velocity error : Sum  Inputs=+-
  Velocity response : Gain  Gain=1/p.ideal.velocityTime
  Zero : Constant  Value=0
  Transmitted force : Outport
  Drive measurements : Outport  Port=2
  wires:
  Acceleration magnitude/1 -> Acceleration limit reached/1
  Acceleration budget/1 -> Acceleration limit reached/2
  [requested_acceleration] -> Acceleration magnitude/1
  Net relative force/1 -> Achieved acceleration/1
  Required axial force/1 -> Available axial force/1, [requested_force_N]
  Ideal capability exceeded/1 -> Effort limit flag/1
  Required force magnitude/1 -> Force limit reached/1
  Force budget/1 -> Force limit reached/2
  Gap position velocity/1 -> Gap motion/1
  [acceleration_limited] -> Ideal capability exceeded/1
  [force_limited] -> Ideal capability exceeded/2
  [ideal_current_A] -> Ideal measurements/1
  [ideal_current_A] -> Ideal measurements/2
  [ideal_current_A] -> Ideal measurements/3
  [ideal_current_A] -> Ideal measurements/4
  [ideal_current_A] -> Ideal measurements/5
  [ideal_effort_limit] -> Ideal measurements/6
  [ideal_current_A] -> Ideal measurements/7
  [ideal_gap_acceleration] -> Ideal measurements/8
  [available_force_N] -> Net relative force/1
  [spring_load_N] -> Net relative force/2
  Command/1 -> Position error/1
  [gap_position_m] -> Position error/2
  Position error/1 -> Position gain/1
  Requested acceleration limit/1 -> Reduced moving mass/1
  Velocity response/1 -> Requested acceleration limit/1, [requested_acceleration]
  Position gain/1 -> Requested speed limit/1
  Reduced moving mass/1 -> Required axial force/1
  [spring_load_N] -> Required axial force/2
  [requested_force_N] -> Required force magnitude/1
  Acceleration limit reached/1 -> [acceleration_limited]
  Available axial force/1 -> [available_force_N], Transmitted force/1
  Force limit reached/1 -> [force_limited]
  Gap motion/1 -> [gap_position_m]
  Gap motion/2 -> [gap_velocity_m_s]
  Zero/1 -> [ideal_current_A]
  Effort limit flag/1 -> [ideal_effort_limit]
  Achieved acceleration/1 -> [ideal_gap_acceleration]
  Spring load/1 -> [spring_load_N]
  Requested speed limit/1 -> Velocity error/1
  [gap_velocity_m_s] -> Velocity error/2
  Velocity error/1 -> Velocity response/1
  Ideal measurements/1 -> Drive measurements/1

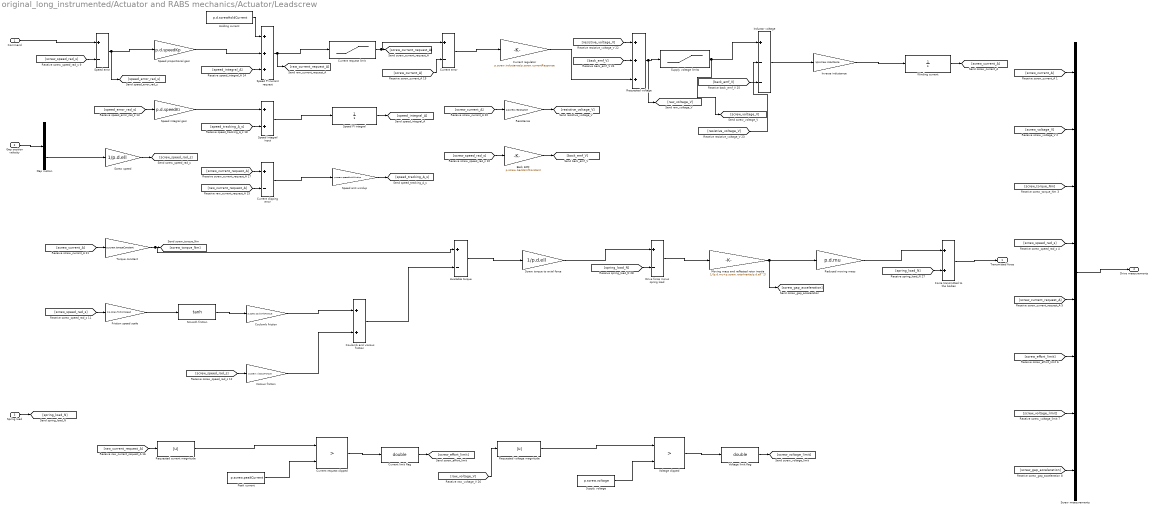
== system original_long_instrumented/Actuator and RABS mechanics/Actuator/Leadscrew ==
  Command : Inport
  Gap position velocity : Inport  Port=2
  Spring load : Inport  Port=3
  Available torque : Sum  Inputs=+-
  Back EMF : Gain  Gain=p.screw.backEmfConstant
  Coulomb and viscous friction : Sum
  Coulomb friction : Gain  Gain=p.screw.coulombTorque
  Current clipping error : Sum  Inputs=+-
  Current error : Sum  Inputs=+-
  Current limit flag : DataTypeConversion  OutDataTypeStr=double  SaturateOnIntegerOverflow=off  RndMeth=Floor
  Current regulator : Gain  Gain=p.screw.inductance/p.screw.currentResponse
  Current request clipped : RelationalOperator  Operator=>  OutDataTypeStr=boolean  RndMeth=Simplest  InputSameDT=off
  Current request limit : Saturate  UpperLimit=p.screw.peakCurrent  LowerLimit=-p.screw.peakCurrent
  Drive force minus spring load : Sum  Inputs=+-
  Force transmitted to the bodies : Sum
  Friction speed scale : Gain  Gain=1/p.screw.frictionSpeed
  Gap motion : Demux  Outputs=2
  Holding current : Constant  Value=p.d.screwHoldCurrent
  Inductor voltage : Sum  Inputs=+--
  Inverse inductance : Gain  Gain=1/p.screw.inductance
  Moving mass and reflected rotor inertia : Gain  Gain=1/(p.d.mu+p.screw.rotorInertia/p.d.ell^2)
  Peak current : Constant  Value=p.screw.peakCurrent
  Reduced moving mass : Gain  Gain=p.d.mu
  Requested current magnitude : Abs  SaturateOnIntegerOverflow=off
  Requested voltage : Sum  Inputs=+++
  Requested voltage magnitude : Abs  SaturateOnIntegerOverflow=off
  Resistance : Gain  Gain=p.screw.resistance
  Screw measurements : Mux  Inputs=8
  Screw speed : Gain  Gain=1/p.d.ell
  Screw torque to axial force : Gain  Gain=1/p.d.ell
  Smooth friction : Trigonometry  Operator=tanh
  Speed PI current request : Sum  Inputs=+++
  Speed PI integral : Integrator
  Speed anti windup : Gain  Gain=p.screw.speedAntiWindup
  Speed error : Sum  Inputs=+-
  Speed integral gain : Gain  Gain=p.d.speedKi
  Speed integral input : Sum
  Speed proportional gain : Gain  Gain=p.d.speedKp
  Supply voltage : Constant  Value=p.screw.voltage
  Supply voltage limits : Saturate  UpperLimit=p.screw.voltage  LowerLimit=-p.screw.voltage
  Torque constant : Gain  Gain=p.screw.torqueConstant
  Viscous friction : Gain  Gain=p.screw.viscousTorque
  Voltage clipped : RelationalOperator  Operator=>  OutDataTypeStr=boolean  RndMeth=Simplest  InputSameDT=off
  Voltage limit flag : DataTypeConversion  OutDataTypeStr=double  SaturateOnIntegerOverflow=off  RndMeth=Floor
  Winding current : Integrator  InitialCondition=p.d.screwHoldCurrent
  Transmitted force : Outport
  Drive measurements : Outport  Port=2
  wires:
  Torque constant/1 -> Available torque/1, [screw_torque_Nm]
  Coulomb and viscous friction/1 -> Available torque/2
  [screw_speed_rad_s] -> Back EMF/1
  Coulomb friction/1 -> Coulomb and viscous friction/1
  Viscous friction/1 -> Coulomb and viscous friction/2
  Smooth friction/1 -> Coulomb friction/1
  [screw_current_request_A] -> Current clipping error/1
  [raw_current_request_A] -> Current clipping error/2
  Current request limit/1 -> Current error/1, [screw_current_request_A]
  [screw_current_A] -> Current error/2
  Current request clipped/1 -> Current limit flag/1
  Current error/1 -> Current regulator/1
  Requested current magnitude/1 -> Current request clipped/1
  Peak current/1 -> Current request clipped/2
  Speed PI current request/1 -> Current request limit/1, [raw_current_request_A]
  Screw torque to axial force/1 -> Drive force minus spring load/1
  [spring_load_N] -> Drive force minus spring load/2
  Reduced moving mass/1 -> Force transmitted to the bodies/1
  [spring_load_N] -> Force transmitted to the bodies/2
  [screw_speed_rad_s] -> Friction speed scale/1
  Gap position velocity/1 -> Gap motion/1
  Supply voltage limits/1 -> Inductor voltage/1, [screw_voltage_V]
  [resistive_voltage_V] -> Inductor voltage/2
  [back_emf_V] -> Inductor voltage/3
  Inductor voltage/1 -> Inverse inductance/1
  Drive force minus spring load/1 -> Moving mass and reflected rotor inertia/1
  Moving mass and reflected rotor inertia/1 -> Reduced moving mass/1, [screw_gap_acceleration]
  [raw_current_request_A] -> Requested current magnitude/1
  [resistive_voltage_V] -> Requested voltage/1
  [back_emf_V] -> Requested voltage/2
  Current regulator/1 -> Requested voltage/3
  [raw_voltage_V] -> Requested voltage magnitude/1
  [screw_current_A] -> Resistance/1
  [screw_current_A] -> Screw measurements/1
  [screw_voltage_V] -> Screw measurements/2
  [screw_torque_Nm] -> Screw measurements/3
  [screw_speed_rad_s] -> Screw measurements/4
  [screw_current_request_A] -> Screw measurements/5
  [screw_effort_limit] -> Screw measurements/6
  [screw_voltage_limit] -> Screw measurements/7
  [screw_gap_acceleration] -> Screw measurements/8
  Gap motion/2 -> Screw speed/1
  Available torque/1 -> Screw torque to axial force/1
  Back EMF/1 -> [back_emf_V]
  Requested voltage/1 -> [raw_voltage_V], Supply voltage limits/1
  Resistance/1 -> [resistive_voltage_V]
  Winding current/1 -> [screw_current_A]
  Current limit flag/1 -> [screw_effort_limit]
  Screw speed/1 -> [screw_speed_rad_s]
  Voltage limit flag/1 -> [screw_voltage_limit]
  Speed error/1 -> [speed_error_rad_s], Speed proportional gain/1
  Speed PI integral/1 -> [speed_integral_A]
  Speed anti windup/1 -> [speed_tracking_A_s]
  Spring load/1 -> [spring_load_N]
  Friction speed scale/1 -> Smooth friction/1
  Holding current/1 -> Speed PI current request/1
  Speed proportional gain/1 -> Speed PI current request/2
  [speed_integral_A] -> Speed PI current request/3
  Speed integral input/1 -> Speed PI integral/1
  Current clipping error/1 -> Speed anti windup/1
  Command/1 -> Speed error/1
  [screw_speed_rad_s] -> Speed error/2
  [speed_error_rad_s] -> Speed integral gain/1
  Speed integral gain/1 -> Speed integral input/1
  [speed_tracking_A_s] -> Speed integral input/2
  [screw_current_A] -> Torque constant/1
  [screw_speed_rad_s] -> Viscous friction/1
  Requested voltage magnitude/1 -> Voltage clipped/1
  Supply voltage/1 -> Voltage clipped/2
  Voltage clipped/1 -> Voltage limit flag/1
  Inverse inductance/1 -> Winding current/1
  Force transmitted to the bodies/1 -> Transmitted force/1
  Screw measurements/1 -> Drive measurements/1
